simulink model "ElectricVehicleThermalManagementWithHeatPump_2026a_version"  (R2026a)
settings: Solver=VariableStepAuto  StopTime=3600  AbsTol=1e-3
PreLoadFcn:
  | init_nmpc
InitFcn:
  | init_nmpc
model workspace: external: MATLAB File ElectricVehicleThermalManagementWithHeatPumpParameters.m (data not in the file)
values from neighbouring files (symbols this model uses):
  battery_C1_LUT = [1913.6 12447 30609 ... (first row only)    [ElectricVehicleThermalManagementWithHeatPumpParameters.m]
  battery_capacity_LUT = [280.081 276.25 276.392]    [ElectricVehicleThermalManagementWithHeatPumpParameters.m]
  battery_cell_cp = 795    [ElectricVehicleThermalManagementWithHeatPumpParameters.m]
  battery_cell_mass = 2.5    [ElectricVehicleThermalManagementWithHeatPumpParameters.m]
  battery_Em_LUT = [3.4966 3.5057 3.5148 ... (first row only)    [ElectricVehicleThermalManagementWithHeatPumpParameters.m]
  battery_N_cells = 20    [ElectricVehicleThermalManagementWithHeatPumpParameters.m]
  battery_Qe_init = 0    [ElectricVehicleThermalManagementWithHeatPumpParameters.m]
  battery_R0_LUT = [0.0117 0.0085 0.009 ... (first row only)    [ElectricVehicleThermalManagementWithHeatPumpParameters.m]
  battery_R1_LUT = [0.0109 0.0029 0.0013 ... (first row only)    [ElectricVehicleThermalManagementWithHeatPumpParameters.m]
  battery_SOC_LUT = [0; 0.1; 0.25; 0.5; 0.75; 0.9; 1]    [ElectricVehicleThermalManagementWithHeatPumpParameters.m]
  battery_T_init = -5    [ElectricVehicleThermalManagementWithHeatPumpParameters.m]
  battery_temperature_LUT = [5 20 40]    [ElectricVehicleThermalManagementWithHeatPumpParameters.m]
  cabin_duct_area = 0.04    [ElectricVehicleThermalManagementWithHeatPumpParameters.m]
  cabin_T_init = -5    [ElectricVehicleThermalManagementWithHeatPumpParameters.m]
  chiller_area_primary = 0.43982297150257105    (= 0.439822971503)    [ElectricVehicleThermalManagementWithHeatPumpParameters.m]
  chiller_N_baffles = 3    [ElectricVehicleThermalManagementWithHeatPumpParameters.m]
  chiller_N_tubes = 100    [ElectricVehicleThermalManagementWithHeatPumpParameters.m]
  chiller_tube_D = 0.0035    [ElectricVehicleThermalManagementWithHeatPumpParameters.m]
  chiller_tube_L = 0.4    [ElectricVehicleThermalManagementWithHeatPumpParameters.m]
  chiller_wall_conductivity = 240    [ElectricVehicleThermalManagementWithHeatPumpParameters.m]
  chiller_wall_thickness = 0.0001    [ElectricVehicleThermalManagementWithHeatPumpParameters.m]
  cond_evap_air_area_flow = 0.3906    [ElectricVehicleThermalManagementWithHeatPumpParameters.m]
  cond_evap_air_area_primary = 1.4834999999999998    (= 1.4835)    [ElectricVehicleThermalManagementWithHeatPumpParameters.m]
  cond_evap_W = 0.015    [ElectricVehicleThermalManagementWithHeatPumpParameters.m]
  cond_evap_wall_conductivity = 240    [ElectricVehicleThermalManagementWithHeatPumpParameters.m]
  cond_evap_wall_thickness = 0.0001    [ElectricVehicleThermalManagementWithHeatPumpParameters.m]
  coolant_channel_D = 0.0092    [ElectricVehicleThermalManagementWithHeatPumpParameters.m]
  coolant_pipe_D = 0.019    [ElectricVehicleThermalManagementWithHeatPumpParameters.m]
  coolant_T_init = -5    [ElectricVehicleThermalManagementWithHeatPumpParameters.m]
  coolant_tank_area = 0.0121    [ElectricVehicleThermalManagementWithHeatPumpParameters.m]
  coolant_tank_volume = 1.25    [ElectricVehicleThermalManagementWithHeatPumpParameters.m]
  coolant_valve_D_ratio_max = 0.95    [ElectricVehicleThermalManagementWithHeatPumpParameters.m]
  coolant_valve_D_ratio_min = 0.001    [ElectricVehicleThermalManagementWithHeatPumpParameters.m]
  coolant_valve_displacement = 0.0063    [ElectricVehicleThermalManagementWithHeatPumpParameters.m]
  coolant_valve_S_max = 0.0053    [ElectricVehicleThermalManagementWithHeatPumpParameters.m]
  evaporator_air_area_flow = 0.12    [ElectricVehicleThermalManagementWithHeatPumpParameters.m]
  evaporator_air_area_primary = 0.4323    [ElectricVehicleThermalManagementWithHeatPumpParameters.m]
  evaporator_W = 0.015    [ElectricVehicleThermalManagementWithHeatPumpParameters.m]
  evaporator_wall_conductivity = 240    [ElectricVehicleThermalManagementWithHeatPumpParameters.m]
  evaporator_wall_thickness = 0.0001    [ElectricVehicleThermalManagementWithHeatPumpParameters.m]
  expansion_valve_D_ratio_max = 0.9    [ElectricVehicleThermalManagementWithHeatPumpParameters.m]
  hex_area_primary = 0.070371675440411369    (= 0.0703716754404)    [ElectricVehicleThermalManagementWithHeatPumpParameters.m]
  hex_N_tubes = 64    [ElectricVehicleThermalManagementWithHeatPumpParameters.m]
  hex_tube_D = 0.0035    [ElectricVehicleThermalManagementWithHeatPumpParameters.m]
  hex_wall_conductivity = 240    [ElectricVehicleThermalManagementWithHeatPumpParameters.m]
  hex_wall_thickness = 0.0001    [ElectricVehicleThermalManagementWithHeatPumpParameters.m]
  inner_cond_air_area_flow = 0.1953    [ElectricVehicleThermalManagementWithHeatPumpParameters.m]
  inner_cond_air_area_primary = 0.99520000000000008    (= 0.9952)    [ElectricVehicleThermalManagementWithHeatPumpParameters.m]
  inner_cond_W = 0.02    [ElectricVehicleThermalManagementWithHeatPumpParameters.m]
  inner_cond_wall_conductivity = 240    [ElectricVehicleThermalManagementWithHeatPumpParameters.m]
  inner_cond_wall_thickness = 0.0001    [ElectricVehicleThermalManagementWithHeatPumpParameters.m]
  pump_speed_max = 1000    [ElectricVehicleThermalManagementWithHeatPumpParameters.m]
  radiator_air_area_flow = 0.097499999999999989    (= 0.0975)    [ElectricVehicleThermalManagementWithHeatPumpParameters.m]
  radiator_air_area_primary = 0.43687499999999996    (= 0.436875)    [ElectricVehicleThermalManagementWithHeatPumpParameters.m]
  radiator_W = 0.015    [ElectricVehicleThermalManagementWithHeatPumpParameters.m]
  radiator_wall_conductivity = 240    [ElectricVehicleThermalManagementWithHeatPumpParameters.m]
  radiator_wall_thickness = 0.0001    [ElectricVehicleThermalManagementWithHeatPumpParameters.m]
  refrigerant_p_init = 0.25    [ElectricVehicleThermalManagementWithHeatPumpParameters.m]
  refrigerant_pipe_D = 0.01    [ElectricVehicleThermalManagementWithHeatPumpParameters.m]
  refrigerant_valve_D_ratio_max = 0.95    [ElectricVehicleThermalManagementWithHeatPumpParameters.m]
  refrigerant_valve_displacement = 0.005    [ElectricVehicleThermalManagementWithHeatPumpParameters.m]
libraries: fl_lib x227, nesl_utility x162, SimscapeFluids_lib x30, LiBatteryElements_lib x16, slpidlib x3, SignalEditorBlockLib x1
(part 5 of 13)

== system ElectricVehicleThermalManagementWithHeatPump_2026a_version/DCDC ==
  Controlled Heat Flow Rate Source : fl_lib/Thermal/Thermal Sources/Controlled Heat Flow Rate Source
  Coolant Jacket : SimscapeFluids_lib/Thermal Liquid/Pipes & Fittings/Pipe (TL)  dynamic_compressibility=simscape.enum.onoff.on  inertia=simscape.enum.onoff.off  num_segments=1  pipe_length=0.2 m  cross_section_geometry=fluids.thermal_liquid.pipes_fittings.enum.CrossSectionGeometry.Custom  pipe_diameter=0.1 m  pipe_inner_diameter=0.05 m  pipe_outer_diameter=0.1 m  pipe_width=0.1 m  pipe_height=0.1 m  pipe_major_axis=0.1 m  pipe_minor_axis=0.05 m  pipe_side=0.1 m  pipe_angle=30 deg  area=pi * coolant_channel_D^2 / 4 m^2  Dh=coolant_channel_D m  annular_heat_transfer_walls=fluids.thermal_liquid.pipes_fittings.enum.AnnularPipeWalls.AnnularInner  elevation_spec=foundation.enum.constant_variable.constant  elevation_gain=0 m  gravity_spec=foundation.enum.constant_variable.constant  g=9.81 m/s^2  pressure_loss_spec=fluids.thermal_liquid.pipes_fittings.enum.PressureLossSpec.Haaland  local_pressure_loss_spec=fluids.thermal_liquid.pipes_fittings.enum.LocalLossSpec.AggregateLength  length_add=0 m  loss_coefficient=0.1  roughness_spec=fluids.thermal_liquid.pipes_fittings.enum.RoughnessSpec.Custom  roughness=1.5e-5 m  Re_friction_TLU=[ 400 1000 1.5e+3 3e+3 4e+3 6e+3 1e+4 2e+4 4e+4 6e+4 1e+5 1e+8 ]  friction_factor_TLU=[ 0.264 0.112 0.07099999999999999 0.0417 0.0387 0.0268 0.025 0.0232 0.0226 0.022 0.0214 0.0214 ]  Re_lam=100  Re_tur=500  shape_factor=64  mdot_nominal=[ 0.1 1 ] kg/s  p_diff_nominal=[ 0.001 0.01 ] MPa  mdot_threshold=1e-6 kg/s  wall_spec=fluids.thermal_liquid.pipes_fittings.enum.wall_spec.rigid  vol_expansion_spec=fluids.thermal_liquid.pipes_fittings.enum.VolumeExpansionSpec.Diameter  area_pressure_gain=1e-6 m^2/MPa  static_pressure_TLU=[.1, 1] MPa  area_pressure_gain_TLU=[1e-05, 1.1e-05] m^2  material_behavior_spec=fluids.thermal_liquid.pipes_fittings.enum.PipeMaterialBehavior.Linear  diameter_pressure_gain=1.2e-6 m/MPa  wall_thickness=0.05 m  elastic_modulus=69 GPa  stress_TLU=[276, 310] MPa  strain_TLU=[.004, .02]  stress_assert_action=simscape.enum.assert.action.none  stress_max=400 MPa  poisson_ratio=0.33  wall_time_constant=0.01 s  environment_spec=foundation.enum.pressure_spec.atmospheric  environment_pressure=0.101325 MPa  thermal_expansion=false  alpha_L_wall=24 um/(deltaK*m)  thermal_expansion_Tref=293.15 K  heat_transfer_spec=fluids.thermal_liquid.pipes_fittings.enum.HeatTransferSpec.DittusBoelter  mdot_nominal_heat=[ 0.1 1 ] kg/s  T_in_nominal=[ 293.15 293.15 ] K  T_out_nominal=[ 300 300 ] K  p_in_nominal_heat=[ 0.101325 0.101325 ] MPa  T_wall_nominal=[ 303.15 303.15 ] K  T_wall_eff_nominal=[303.15, 303.15] K  a_coeff=0.3  b_Re_power=0.8  c_Pr_power=0.33  Nu_lam=3.66  Re_Colburn_TLU=[ 100 150 1000 ]  Colburn_factor_TLU=[ 0.019 0.013 0.002 ]  Re_Nu_TLU=[ 100 150 1000 ]  Pr_Nu_TLU=[ 1 10 ]  Nu_TLU=[ 3.72 4.21; 3.75 4.44; 4.21 7.15 ]  annular_correction=fluids.thermal_liquid.pipes_fittings.enum.AnnularPipeCorrectionFactor.Gnielinski  p0_vec=coolant_p_init MPa  T0_vec=coolant_T_init degC  mdot0=0.1 kg/s  p_nominal=0.101325 MPa  T_nominal=293.15 K
  DC-DC Converter : fl_lib/Thermal/Thermal Elements/Thermal Mass  mass_type=foundation.enum.constant_variable.constant  mass=1 kg  sp_heat=447 J/kg/K  mass_min=1e-6 kg  num_ports=foundation.enum.numPorts2.one  m_specify=off  m_priority=High  m=1 kg  m_nominal_specify=off  m_nominal_value=1  m_nominal_unit=kg  T_specify=on  T_priority=High  T=coolant_T_init degC  T_nominal_specify=off  T_nominal_value=1  T_nominal_unit=K  Q_specify=off  Q_priority=None  Q=0 W  Q_nominal_specify=off  Q_nominal_value=1  Q_nominal_unit=W
  Flow Rate Sensor (TL) : fl_lib/Thermal Liquid/Sensors/Flow Rate Sensor (TL)  mass_flow_measure=true  volumetric_flow_measure=false  energy_flow_measure=true
  Flow Resistance (TL) : fl_lib/Thermal Liquid/Elements/Flow Resistance (TL)  delta_p_nominal=2e-3 MPa  mdot_nominal=0.02 kg/s  area=pi * coolant_pipe_D^2 / 4 m^2  laminar_fraction=1e-3
  Flow Resistance (TL)1 : fl_lib/Thermal Liquid/Elements/Flow Resistance (TL)  delta_p_nominal=1e-5 MPa  mdot_nominal=0.02 kg/s  area=pi * coolant_pipe_D^2 / 4 m^2  laminar_fraction=1e-3
  PS-Simulink Converter : nesl_utility/PS-Simulink Converter  PhysicalDomain=network_engine_domain  SubClassName=ps_output  LeftPortType=input  RightPortType=output  PseudoPeriodic=off  Frequencies=[]  VectorFormat=inherit  Unit=degC  AffineConversion=on
  PS-Simulink Converter1 : nesl_utility/PS-Simulink Converter  PhysicalDomain=network_engine_domain  SubClassName=ps_output  LeftPortType=input  RightPortType=output  PseudoPeriodic=off  Frequencies=[]  VectorFormat=inherit  Unit=inherit  AffineConversion=off
  Scope : Scope
      settings: ActiveDisplayYMinimum=-0.0018  ActiveDisplayYMaximum=0.01621  DataLoggingVariableName=ScopeData8
  Simulink-PS Converter : nesl_utility/Simulink-PS Converter  PhysicalDomain=network_engine_domain  SubClassName=ps_input  LeftPortType=input  RightPortType=output  PseudoPeriodic=off  Frequencies=[]  NoiseDistribution=none  NoiseParameters=[]  Unit=W  AffineConversion=off  FilteringAndDerivatives=provide  SimscapeFilterOrder=1  InputFilterTimeConstant=0.001  UdotUserProvided=0
  Temperature Sensor : fl_lib/Thermal/Thermal Sensors/Temperature Sensor  temperature_measure=foundation.enum.MeasurementReference.absolute
  Thermal Reference : fl_lib/Thermal/Thermal Elements/Thermal Reference
  To Workspace : ToWorkspace  VariableName=mf_dcdc  SampleTime=-1
  To Workspace1 : ToWorkspace  VariableName=Q_dcdcMeasured  SampleTime=-1
  To Workspace2 : ToWorkspace  VariableName=T_dcdcMeas  SampleTime=-1
  B : PMIOPort  Side=Left
  A : PMIOPort  Port=2  Side=Right
  tag scope: T_dcdc=global
  wires:
  [Q_dcdc] -> To Workspace1/1, Simulink-PS Converter/1
  PS-Simulink Converter/1 -> To Workspace2/1, [T_dcdc]
  PS-Simulink Converter1/1 -> To Workspace/1, Scope/1
  connections:
  Coolant Jacket/LConn2 -- Controlled Heat Flow Rate Source/LConn1 -- Temperature Sensor/LConn1 -- DC-DC Converter/LConn1
  PS-Simulink Converter/LConn1 -- Temperature Sensor/RConn1
  Controlled Heat Flow Rate Source/RConn2 -- Thermal Reference/LConn1
  Simulink-PS Converter/RConn1 -- Controlled Heat Flow Rate Source/RConn1
  Coolant Jacket/LConn1 -- Flow Rate Sensor (TL)/RConn1
  PS-Simulink Converter1/LConn1 -- Flow Rate Sensor (TL)/RConn2
  Flow Resistance (TL)/LConn1 -- A/RConn1
  Flow Resistance (TL)/RConn1 -- Flow Rate Sensor (TL)/LConn1
  Flow Resistance (TL)1/LConn1 -- Coolant Jacket/RConn1
  Flow Resistance (TL)1/RConn1 -- B/RConn1

== system ElectricVehicleThermalManagementWithHeatPump_2026a_version/Evaporator ==
  Evaporator : SimscapeFluids_lib/Heat Exchangers/Two-Phase Fluid - Moist Air/Condenser Evaporator (2P-MA)  flow_arrangement=fluids.heat_exchangers.enum.FlowArrangement2PMA.Cross  cross_flow_arrangement=fluids.heat_exchangers.enum.CrossFlowArrangement2PMA.UnmixedUnmixed  R_wall=evaporator_wall_thickness / evaporator_air_area_primary / evaporator_wall_conductivity K/W  wall_thermal_mass=false  mass_wall=1 kg  cp_wall=490 J/(K*kg)  area_A1=pi * refrigerant_pipe_D^2 / 4 m^2  area_B1=pi * refrigerant_pipe_D^2 / 4 m^2  area_A2=cabin_duct_area m^2  area_B2=cabin_duct_area m^2  tube_num_2P=evaporator_N_tubes  tube_length_2P=evaporator_L m  tube_cross_section_2P=fluids.heat_exchangers.enum.TubeCrossSection.Rectangular  tube_diameter_2P=0.1 m  tube_width_2P=evaporator_W m  tube_height_2P=evaporator_tube_H m  tube_inner_diameter_2P=0.05 m  tube_outer_diameter_2P=0.1 m  tube_flow_area_2P=0.01 m^2  tube_wetted_perimeter_2P=0.4 m  tube_heat_perimeter_2P=0.4 m  tube_pressure_loss_spec_2P=fluids.heat_exchangers.enum.TubePressureLossSpec2P.Haaland  tube_loss_coeff_2P=10  tube_local_pressure_loss_spec_2P=fluids.heat_exchangers.enum.LocalLossSpec.AggregateLength  tube_length_add_2P=evaporator_tube_Leq m  tube_local_loss_coefficient_2P=0.1  tube_roughness_pressure_2P=15e-6 m  tube_Re_lam_pressure_2P=2000  tube_Re_tur_pressure_2P=4000  tube_shape_factor_generic_2P=64  tube_heat_coeff_spec_2P=fluids.heat_exchangers.enum.TubeHeatCoeffSpec2P.GneilinskiCavalliniZecchin  tube_colburn_coeff_liq_2P=[.023, .8, .33]  tube_colburn_coeff_mix_2P=[.05, .8, .33]  tube_colburn_coeff_vap_2P=[.023, .8, .33]  tube_roughness_heat_2P=15e-6 m  tube_Re_lam_heat_2P=2000  tube_Re_tur_heat_2P=4000  tube_Nu_lam_generic_2P=3.66  fouling_factor_2P=0.1 m^2*K/kW  fin_area_2P=evaporator_tube_area_webs m^2  fin_efficiency_2P=0.6  energy_spec_2P=foundation.enum.energy_spec.void_fraction  p_init_2P=refrigerant_p_init MPa  T_init_2P=293.15 K  x_init_2P=0.5  alpha_init_2P=refrigerant_alpha_init  h_init_2P=1500 kJ/kg  u_init_2P=1500 kJ/kg  flow_geometry_MA=fluids.heat_exchangers.enum.FlowGeometryMA.Generic  tube_num_MA=1  tube_length_MA=5 m  tube_cross_section_MA=fluids.heat_exchangers.enum.TubeCrossSection.Circular  tube_diameter_MA=0.1 m  tube_width_MA=0.1 m  tube_height_MA=0.1 m  tube_inner_diameter_MA=0.05 m  tube_outer_diameter_MA=0.1 m  tube_flow_area_MA=0.01 m^2  tube_wetted_perimeter_MA=0.4 m  tube_heat_perimeter_MA=0.4 m  tube_pressure_loss_spec_MA=fluids.heat_exchangers.enum.TubePressureLossSpec.Haaland  tube_loss_coeff_MA=10  tube_local_pressure_loss_spec_MA=fluids.heat_exchangers.enum.LocalLossSpec.AggregateLength  tube_length_add_MA=0.1 m  tube_local_loss_coefficient_MA=0.1  tube_roughness_pressure_MA=15e-6 m  tube_Re_lam_pressure_MA=2000  tube_Re_tur_pressure_MA=4000  tube_shape_factor_generic_MA=64  tube_heat_coeff_spec_MA=fluids.heat_exchangers.enum.TubeHeatCoeffSpec.Gneilinski  tube_colburn_coeff_MA=[.023, .8, .33]  tube_roughness_heat_MA=15e-6 m  tube_Re_lam_heat_MA=2000  tube_Re_tur_heat_MA=4000  tube_Nu_lam_generic_MA=3.66  bank_arrangement_MA=fluids.heat_exchangers.enum.BankArrangement.Inline  bank_num_rows_MA=5  bank_tubes_per_row_MA=5  bank_width_MA=1 m  bank_tube_diameter_MA=0.05 m  bank_longitudinal_pitch_MA=0.15 m  bank_transverse_pitch_MA=0.15 m  bank_pressure_loss_spec_MA=fluids.heat_exchangers.enum.BankPressureLossSpec.Martin  bank_euler_MA=10  bank_heat_coeff_spec_MA=fluids.heat_exchangers.enum.BankHeatCoeffSpec.Martin  bank_colburn_coeff_MA=[.27, .63, .36]  generic_flow_area_MA=evaporator_air_area_flow m^2  generic_heat_area_MA=evaporator_air_area_primary m^2  generic_volume_MA=evaporator_air_area_flow * evaporator_W m^3  generic_loss_coeff_MA=10  generic_colburn_coeff_MA=[0.27, 0.63, 0.36]  fouling_factor_MA=0.1 m^2*K/kW  fin_area_MA=evaporator_air_area_fins m^2  fin_efficiency_MA=0.7  p_init_MA=cabin_p_init MPa  T_init_MA=cabin_T_init degC  humidity_spec_MA=foundation.enum.HumiditySpec.RelativeHumidity  RH_init_MA=cabin_RH_init  x_w_init_MA=0.01  y_w_init_MA=0.01  HR_init_MA=0.01  Tw_init_MA=287 K  trace_gas_spec_MA=foundation.enum.trace_gas_spec.mole_fraction  x_g_init_MA=0.001  y_g_init_MA=cabin_CO2_init  r_d_init_MA=0  RH_ws_MA=1  time_constant_cond_MA=1e-3 s  time_constant_evap_MA=1e-3 s  fraction_entrained_MA=1
  Flow Resistance (2P) : fl_lib/Two-Phase Fluid/Elements/Flow Resistance (2P)  delta_p_nominal=1e-4 MPa  mdot_nominal=0.01 kg/s  v_nominal=0 m^3/kg  area=pi * refrigerant_pipe_D^2 / 4 m^2  laminar_fraction=1e-3
  PS-Simulink Converter{,1..3} (4 alike) : nesl_utility/PS-Simulink Converter  PhysicalDomain=network_engine_domain  SubClassName=ps_output  LeftPortType=input  RightPortType=output  PseudoPeriodic=off  Frequencies=[]  VectorFormat=inherit  Unit=inherit  AffineConversion=off
  Pressure & Temperature Sensor (MA) : fl_lib/Moist Air/Sensors/Pressure & Temperature Sensor (MA)  reference=foundation.enum.MeasurementReference.absolute  pressure=true  pressure_spec=foundation.enum.PressureMeasementSpec.Absolute  temperature=true
  Pressure & Temperature Sensor (MA)1 : fl_lib/Moist Air/Sensors/Pressure & Temperature Sensor (MA)  reference=foundation.enum.MeasurementReference.absolute  pressure=true  pressure_spec=foundation.enum.PressureMeasementSpec.Absolute  temperature=true
  SR7 : Subsystem
  SR8 : Subsystem
  Scope : Scope
      settings: ActiveDisplayYMinimum=254.07357  ActiveDisplayYMaximum=301.11104  DataLoggingVariableName=ScopeData3
  To Workspace : ToWorkspace  VariableName=airEvapPressure_out  SampleTime=-1
  To Workspace1 : ToWorkspace  VariableName=airEvapTemp_out  SampleTime=-1
  To Workspace2 : ToWorkspace  VariableName=airEvapPressure_in  SampleTime=-1
  To Workspace3 : ToWorkspace  VariableName=airEvapTemp_in  SampleTime=-1
  A : PMIOPort  Side=Left
  D : PMIOPort  Port=2  Side=Left
  B : PMIOPort  Port=3  Side=Right
  C : PMIOPort  Port=4  Side=Right
  wires:
  PS-Simulink Converter/1 -> To Workspace/1
  PS-Simulink Converter3/1 -> Scope/1, To Workspace1/1
  PS-Simulink Converter1/1 -> To Workspace2/1
  PS-Simulink Converter2/1 -> To Workspace3/1
  connections:
  SR8/LConn1 -- Evaporator/LConn3
  SR7/RConn1 -- Evaporator/LConn1
  SR8/RConn1 -- Flow Resistance (2P)/LConn1
  Evaporator/RConn3 -- Pressure & Temperature Sensor (MA)1/LConn1 -- C/RConn1
  Flow Resistance (2P)/RConn1 -- B/RConn1
  Evaporator/RConn1 -- D/RConn1 -- Pressure & Temperature Sensor (MA)/LConn1
  SR7/LConn1 -- A/RConn1
  PS-Simulink Converter/LConn1 -- Pressure & Temperature Sensor (MA)/RConn1
  PS-Simulink Converter1/LConn1 -- Pressure & Temperature Sensor (MA)1/RConn1
  PS-Simulink Converter2/LConn1 -- Pressure & Temperature Sensor (MA)1/RConn2
  PS-Simulink Converter3/LConn1 -- Pressure & Temperature Sensor (MA)/RConn2

== system ElectricVehicleThermalManagementWithHeatPump_2026a_version/Evaporator Expansion Valve ==
  Evaporator Expansion Valve : SimscapeFluids_lib/Two-Phase Fluid/Valves & Orifices/Orifice (2P)  orifice_type=foundation.enum.constant_variable.variable  constant_liquid_orifice_parameterization=fluids.two_phase_fluid.valves_orifices.enum.LiquidConstantOrificeParameterization.Area  variable_liquid_orifice_parameterization=fluids.two_phase_fluid.valves_orifices.enum.LiquidOrificeParameterization.LinearArea  mdot_nominal_constant=0.1 kg/s  delta_p_nominal_constant=0.001 MPa  orifice_area_constant=1e-4 m^2  S_min=0 m  del_S=refrigerant_valve_displacement m  open_orientation=fluids.two_phase_fluid.valves_orifices.enum.OrificeOrientation.Positive  mdot_nominal_max=0.1 kg/s  delta_p_nominal_max=0.001 MPa  orifice_area_max=pi * (expansion_valve_D_ratio_max*refrigerant_pipe_D)^2 / 4 m^2  S_TLU=[0, .002, .004, .007, .017] m  orifice_area_TLU=[1e-10, 2e-05, 4e-05, 6e-05, 8e-05, .0001] m^2  energy_spec=foundation.enum.energy_spec.temperature  p_inlet=0.101325 MPa  T_inlet=293.15 K  x_inlet=0  alpha_inlet=0  h_inlet=400 kJ/kg  u_inlet=400 kJ/kg  Cd=0.7  pressure_recovery=true  leakage_fraction=1e-6  smoothing_factor=0.01  B_lam=0.999  tau_x=0.1 s  area=pi * refrigerant_pipe_D^2 / 4 m^2  vapor_orifice_parameterization=fluids.two_phase_fluid.valves_orifices.enum.VaporOrificeParameterization.Cv  opening_characteristic=fluids.two_phase_fluid.valves_orifices.enum.OpeningCharacteristics.Linear  Cv_constant=4  Cv_max=4  S_Cv_TLU=[0, .003, .006, .009, .012, .015] m  Cv_TLU=[1e-06, .8, 1.6, 2.4, 3.2, 4]  xT_Cv=0.7  Kv_constant=3.6  Kv_max=3.6  S_Kv_TLU=[0, .003, .006, .009, .012, .015] m  Kv_TLU=[1e-06, .72, 1.44, 2.16, 2.88, 3.6]  xT_Kv=0.7  S_orifice_area_TLU=[0, .003, .006, .009, .012, .015] m
  Max Valve Displacement [m] : Gain  Gain=refrigerant_valve_displacement
  Simulink-PS Converter : nesl_utility/Simulink-PS Converter  PhysicalDomain=network_engine_domain  SubClassName=ps_input  LeftPortType=input  RightPortType=output  PseudoPeriodic=off  Frequencies=[]  NoiseDistribution=none  NoiseParameters=[]  Unit=m  AffineConversion=off  FilteringAndDerivatives=provide  SimscapeFilterOrder=1  InputFilterTimeConstant=0.001  UdotUserProvided=0
  Transfer Fcn : TransferFcn  Denominator=[1 1]
  A : PMIOPort  Side=Left
  B : PMIOPort  Port=2  Side=Right
  wires:
  Transfer Fcn/1 -> Max Valve Displacement [m]/1
  [cmd_exv_evap] -> Transfer Fcn/1
  Max Valve Displacement [m]/1 -> Simulink-PS Converter/1
  connections:
  Evaporator Expansion Valve/LConn2 -- Simulink-PS Converter/RConn1
  Evaporator Expansion Valve/LConn1 -- A/RConn1
  Evaporator Expansion Valve/RConn1 -- B/RConn1

== system ElectricVehicleThermalManagementWithHeatPump_2026a_version/Heat Exchanger ==
  Flow Rate Sensor (TL) : fl_lib/Thermal Liquid/Sensors/Flow Rate Sensor (TL)  mass_flow_measure=true  volumetric_flow_measure=false  energy_flow_measure=true
  Heat Exchanger : SimscapeFluids_lib/Heat Exchangers/Two-Phase Fluid - Thermal Liquid/Condenser Evaporator (TL-2P)  flow_arrangement=fluids.heat_exchangers.enum.FlowArrangementTL2P.Cross  cross_flow_arrangement=fluids.heat_exchangers.enum.CrossFlowArrangementTL2P.UnmixedMixed  R_wall=hex_wall_thickness / hex_area_primary / hex_wall_conductivity K/W  wall_thermal_mass=false  mass_wall=1 kg  cp_wall=490 J/(K*kg)  area_A1=pi * coolant_pipe_D^2 / 4 m^2  area_B1=pi * coolant_pipe_D^2 / 4 m^2  area_A2=pi * refrigerant_pipe_D^2 / 4 m^2  area_B2=pi * refrigerant_pipe_D^2 / 4 m^2  flow_geometry_TL=fluids.heat_exchangers.enum.FlowGeometryTL.AcrossTubeBank  tube_num_TL=1  tube_length_TL=5 m  tube_cross_section_TL=fluids.heat_exchangers.enum.TubeCrossSection.Circular  tube_diameter_TL=0.1 m  tube_width_TL=0.1 m  tube_height_TL=0.1 m  tube_inner_diameter_TL=0.05 m  tube_outer_diameter_TL=0.1 m  tube_flow_area_TL=0.01 m^2  tube_wetted_perimeter_TL=0.4 m  tube_heat_perimeter_TL=0.4 m  tube_pressure_loss_spec_TL=fluids.heat_exchangers.enum.TubePressureLossSpec.Haaland  tube_loss_coeff_TL=10  tube_local_pressure_loss_spec_TL=fluids.heat_exchangers.enum.LocalLossSpec.AggregateLength  tube_length_add_TL=0.1 m  tube_local_loss_coefficient_TL=0.1  tube_roughness_pressure_TL=15e-6 m  tube_Re_lam_pressure_TL=2000  tube_Re_tur_pressure_TL=4000  tube_shape_factor_generic_TL=64  tube_heat_coeff_spec_TL=fluids.heat_exchangers.enum.TubeHeatCoeffSpec.Gneilinski  tube_colburn_coeff_TL=[.023, .8, .33]  tube_roughness_heat_TL=15e-6 m  tube_Re_lam_heat_TL=2000  tube_Re_tur_heat_TL=4000  tube_Nu_lam_generic_TL=3.66  bank_arrangement_TL=fluids.heat_exchangers.enum.BankArrangement.Staggered  bank_num_rows_TL=sqrt(hex_N_tubes)  bank_tubes_per_row_TL=sqrt(hex_N_tubes)  bank_width_TL=hex_tube_L m  bank_tube_diameter_TL=hex_tube_D m  bank_longitudinal_pitch_TL=2 * hex_tube_D m  bank_transverse_pitch_TL=2 * hex_tube_D m  bank_pressure_loss_spec_TL=fluids.heat_exchangers.enum.BankPressureLossSpec.Martin  bank_euler_TL=10  bank_heat_coeff_spec_TL=fluids.heat_exchangers.enum.BankHeatCoeffSpec.Martin  bank_colburn_coeff_TL=[.27, .63, .36]  generic_flow_area_TL=0.01 m^2  generic_heat_area_TL=2 m^2  generic_volume_TL=0.05 m^3  generic_loss_coeff_TL=10  generic_colburn_coeff_TL=[.023, .8, .33]  fouling_factor_TL=0.1 m^2*K/kW  fin_area_TL=0 m^2  fin_efficiency_TL=0  p_init_TL=coolant_p_init MPa  T_init_TL=coolant_T_init degC  tube_num_2P=hex_N_tubes  tube_length_2P=hex_tube_L m  tube_cross_section_2P=fluids.heat_exchangers.enum.TubeCrossSection.Circular  tube_diameter_2P=hex_tube_D m  tube_width_2P=0.1 m  tube_height_2P=0.1 m  tube_inner_diameter_2P=0.05 m  tube_outer_diameter_2P=0.1 m  tube_flow_area_2P=0.01 m^2  tube_wetted_perimeter_2P=0.4 m  tube_heat_perimeter_2P=0.4 m  tube_pressure_loss_spec_2P=fluids.heat_exchangers.enum.TubePressureLossSpec2P.Haaland  tube_loss_coeff_2P=10  tube_local_pressure_loss_spec_2P=fluids.heat_exchangers.enum.LocalLossSpec.AggregateLength  tube_length_add_2P=hex_tube_Leq m  tube_local_loss_coefficient_2P=0.1  tube_roughness_pressure_2P=15e-6 m  tube_Re_lam_pressure_2P=2000  tube_Re_tur_pressure_2P=4000  tube_shape_factor_generic_2P=64  tube_heat_coeff_spec_2P=fluids.heat_exchangers.enum.TubeHeatCoeffSpec2P.GneilinskiCavalliniZecchin  tube_colburn_coeff_liq_2P=[.023, .8, .33]  tube_colburn_coeff_mix_2P=[.05, .8, .33]  tube_colburn_coeff_vap_2P=[.023, .8, .33]  tube_roughness_heat_2P=15e-6 m  tube_Re_lam_heat_2P=2000  tube_Re_tur_heat_2P=4000  tube_Nu_lam_generic_2P=3.66  fouling_factor_2P=0.1 m^2*K/kW  fin_area_2P=0 m^2  fin_efficiency_2P=0  energy_spec_2P=foundation.enum.energy_spec.void_fraction  p_init_2P=refrigerant_p_init MPa  T_init_2P=293.15 K  x_init_2P=0.5  alpha_init_2P=refrigerant_alpha_init  h_init_2P=1500 kJ/kg  u_init_2P=1500 kJ/kg
  PS-Simulink Converter : nesl_utility/PS-Simulink Converter  PhysicalDomain=network_engine_domain  SubClassName=ps_output  LeftPortType=input  RightPortType=output  PseudoPeriodic=off  Frequencies=[]  VectorFormat=inherit  Unit=inherit  AffineConversion=off
  PS-Simulink Converter1 : nesl_utility/PS-Simulink Converter  PhysicalDomain=network_engine_domain  SubClassName=ps_output  LeftPortType=input  RightPortType=output  PseudoPeriodic=off  Frequencies=[]  VectorFormat=inherit  Unit=inherit  AffineConversion=off
  PS-Simulink Converter2 : nesl_utility/PS-Simulink Converter  PhysicalDomain=network_engine_domain  SubClassName=ps_output  LeftPortType=input  RightPortType=output  PseudoPeriodic=off  Frequencies=[]  VectorFormat=inherit  Unit=inherit  AffineConversion=off
  Pressure & Temperature Sensor (TL) : fl_lib/Thermal Liquid/Sensors/Pressure & Temperature Sensor (TL)  reference=foundation.enum.MeasurementReference.absolute  pressure=false  pressure_spec=foundation.enum.PressureMeasementSpec.Absolute  temperature=true
  Pressure & Temperature Sensor (TL)1 : fl_lib/Thermal Liquid/Sensors/Pressure & Temperature Sensor (TL)  reference=foundation.enum.MeasurementReference.absolute  pressure=false  pressure_spec=foundation.enum.PressureMeasementSpec.Absolute  temperature=true
  SR5 : Subsystem
  SR6 : Subsystem
  Scope : Scope
      settings: ActiveDisplayYMinimum=256.69677  ActiveDisplayYMaximum=319.19994  DataLoggingVariableName=ScopeData2
  Scope1 : Scope
      settings: ActiveDisplayYMinimum=252.53888  ActiveDisplayYMaximum=358.65007  DataLoggingVariableName=ScopeData3
  Scope2 : Scope
      settings: ActiveDisplayYMinimum=-0.04462  ActiveDisplayYMaximum=0.40154
  To Workspace : ToWorkspace  VariableName=heatExchangerCoolantT_outK  SampleTime=-1
  To Workspace1 : ToWorkspace  VariableName=heatExchangerCoolantT_inK  SampleTime=-1
  To Workspace2 : ToWorkspace  VariableName=mf_htxClnt  SampleTime=-1
  D : PMIOPort  Side=Left
  A : PMIOPort  Port=2  Side=Left
  C : PMIOPort  Port=3  Side=Right
  B : PMIOPort  Port=4  Side=Right
  wires:
  PS-Simulink Converter/1 -> To Workspace/1, Scope/1
  PS-Simulink Converter1/1 -> Scope1/1, To Workspace1/1
  PS-Simulink Converter2/1 -> To Workspace2/1, Scope2/1
  connections:
  Heat Exchanger/RConn2 -- SR6/LConn1
  SR6/RConn1 -- B/RConn1
  Heat Exchanger/RConn1 -- SR5/RConn1
  SR5/LConn1 -- A/RConn1
  C/RConn1 -- Pressure & Temperature Sensor (TL)1/LConn1 -- Heat Exchanger/LConn2
  Pressure & Temperature Sensor (TL)/LConn1 -- D/RConn1 -- Flow Rate Sensor (TL)/RConn1
  PS-Simulink Converter/LConn1 -- Pressure & Temperature Sensor (TL)/RConn1
  PS-Simulink Converter1/LConn1 -- Pressure & Temperature Sensor (TL)1/RConn1
  PS-Simulink Converter2/LConn1 -- Flow Rate Sensor (TL)/RConn2
  Flow Rate Sensor (TL)/LConn1 -- Heat Exchanger/LConn1

== system ElectricVehicleThermalManagementWithHeatPump_2026a_version/Heat Pump Expansion Valve ==
  Heat Pump Expansion Valve : SimscapeFluids_lib/Two-Phase Fluid/Valves & Orifices/Orifice (2P)  orifice_type=foundation.enum.constant_variable.variable  constant_liquid_orifice_parameterization=fluids.two_phase_fluid.valves_orifices.enum.LiquidConstantOrificeParameterization.Area  variable_liquid_orifice_parameterization=fluids.two_phase_fluid.valves_orifices.enum.LiquidOrificeParameterization.LinearArea  mdot_nominal_constant=0.1 kg/s  delta_p_nominal_constant=0.001 MPa  orifice_area_constant=1e-4 m^2  S_min=0 m  del_S=refrigerant_valve_displacement m  open_orientation=fluids.two_phase_fluid.valves_orifices.enum.OrificeOrientation.Positive  mdot_nominal_max=0.1 kg/s  delta_p_nominal_max=0.001 MPa  orifice_area_max=pi * (expansion_valve_D_ratio_max*refrigerant_pipe_D)^2 / 4 m^2  S_TLU=[0, .002, .004, .007, .017] m  orifice_area_TLU=[1e-10, 2e-05, 4e-05, 6e-05, 8e-05, .0001] m^2  energy_spec=foundation.enum.energy_spec.temperature  p_inlet=0.101325 MPa  T_inlet=293.15 K  x_inlet=0  alpha_inlet=0  h_inlet=400 kJ/kg  u_inlet=400 kJ/kg  Cd=0.7  pressure_recovery=true  leakage_fraction=1e-6  smoothing_factor=0.01  B_lam=0.999  tau_x=0.1 s  area=pi * refrigerant_pipe_D^2 / 4 m^2  vapor_orifice_parameterization=fluids.two_phase_fluid.valves_orifices.enum.VaporOrificeParameterization.Cv  opening_characteristic=fluids.two_phase_fluid.valves_orifices.enum.OpeningCharacteristics.Linear  Cv_constant=4  Cv_max=4  S_Cv_TLU=[0, .003, .006, .009, .012, .015] m  Cv_TLU=[1e-06, .8, 1.6, 2.4, 3.2, 4]  xT_Cv=0.7  Kv_constant=3.6  Kv_max=3.6  S_Kv_TLU=[0, .003, .006, .009, .012, .015] m  Kv_TLU=[1e-06, .72, 1.44, 2.16, 2.88, 3.6]  xT_Kv=0.7  S_orifice_area_TLU=[0, .003, .006, .009, .012, .015] m
  Max Valve Displacement [m] : Gain  Gain=refrigerant_valve_displacement
  PS-Simulink Converter : nesl_utility/PS-Simulink Converter  PhysicalDomain=network_engine_domain  SubClassName=ps_output  LeftPortType=input  RightPortType=output  PseudoPeriodic=off  Frequencies=[]  VectorFormat=inherit  Unit=inherit  AffineConversion=off
  PS-Simulink Converter1 : nesl_utility/PS-Simulink Converter  PhysicalDomain=network_engine_domain  SubClassName=ps_output  LeftPortType=input  RightPortType=output  PseudoPeriodic=off  Frequencies=[]  VectorFormat=inherit  Unit=inherit  AffineConversion=off
  "Pressure, Temperature & Internal Energy Sensor (2P)" : fl_lib/Two-Phase Fluid/Sensors/Pressure, Temperature & Internal Energy Sensor (2P)  reference=foundation.enum.MeasurementReference.absolute  pressure=true  pressure_spec=foundation.enum.PressureMeasementSpec.Absolute  temperature=false  internal_energy=false
  "Pressure, Temperature & Internal Energy Sensor (2P)1" : fl_lib/Two-Phase Fluid/Sensors/Pressure, Temperature & Internal Energy Sensor (2P)  reference=foundation.enum.MeasurementReference.absolute  pressure=true  pressure_spec=foundation.enum.PressureMeasementSpec.Absolute  temperature=false  internal_energy=false
  Scope : Scope
      settings: ActiveDisplayYMinimum=-4E-6  ActiveDisplayYMaximum=3.9E-5
  Simulink-PS Converter : nesl_utility/Simulink-PS Converter  PhysicalDomain=network_engine_domain  SubClassName=ps_input  LeftPortType=input  RightPortType=output  PseudoPeriodic=off  Frequencies=[]  NoiseDistribution=none  NoiseParameters=[]  Unit=m  AffineConversion=off  FilteringAndDerivatives=provide  SimscapeFilterOrder=1  InputFilterTimeConstant=0.001  UdotUserProvided=0
  To Workspace : ToWorkspace  VariableName=EXVRefPress_inMpa  SampleTime=-1
  To Workspace1 : ToWorkspace  VariableName=EXVRefPress_outMpa  SampleTime=-1
  Transfer Fcn : TransferFcn  Denominator=[1 1]
  B : PMIOPort  Side=Left
  A : PMIOPort  Port=2  Side=Right
  wires:
  Max Valve Displacement [m]/1 -> Scope/1, Simulink-PS Converter/1
  [cmd_exv_heatpump] -> Transfer Fcn/1
  Transfer Fcn/1 -> Max Valve Displacement [m]/1
  PS-Simulink Converter/1 -> To Workspace/1
  PS-Simulink Converter1/1 -> To Workspace1/1
  connections:
  Heat Pump Expansion Valve/RConn1 -- "Pressure, Temperature & Internal Energy Sensor (2P)1"/LConn1 -- B/RConn1
  Heat Pump Expansion Valve/LConn1 -- "Pressure, Temperature & Internal Energy Sensor (2P)"/LConn1 -- A/RConn1
  Heat Pump Expansion Valve/LConn2 -- Simulink-PS Converter/RConn1
  PS-Simulink Converter/LConn1 -- "Pressure, Temperature & Internal Energy Sensor (2P)"/RConn1
  PS-Simulink Converter1/LConn1 -- "Pressure, Temperature & Internal Energy Sensor (2P)1"/RConn1

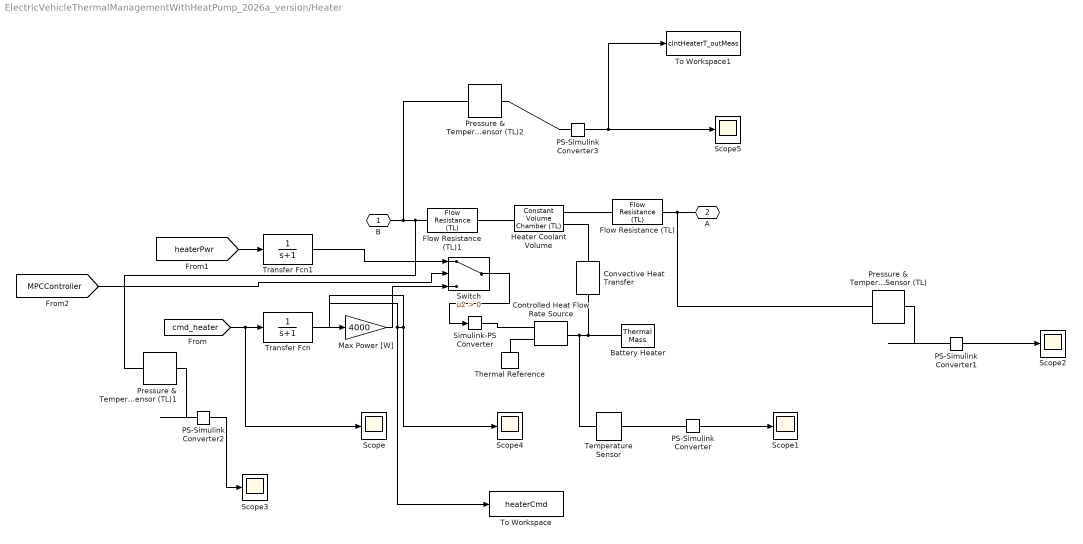
== system ElectricVehicleThermalManagementWithHeatPump_2026a_version/Heater ==
  Battery Heater : fl_lib/Thermal/Thermal Elements/Thermal Mass  mass_type=foundation.enum.constant_variable.constant  mass=2 kg  sp_heat=447 J/kg/K  mass_min=1e-6 kg  num_ports=foundation.enum.numPorts2.one  m_specify=off  m_priority=High  m=1 kg  m_nominal_specify=off  m_nominal_value=1  m_nominal_unit=kg  T_specify=on  T_priority=High  T=coolant_T_init degC  T_nominal_specify=off  T_nominal_value=1  T_nominal_unit=K  Q_specify=off  Q_priority=None  Q=0 W  Q_nominal_specify=off  Q_nominal_value=1  Q_nominal_unit=W
  Controlled Heat Flow Rate Source : fl_lib/Thermal/Thermal Sources/Controlled Heat Flow Rate Source
  Convective Heat Transfer : fl_lib/Thermal/Thermal Elements/Convective Heat Transfer  thermal_type=foundation.enum.constant_variable.constant  area=1 m^2  heat_tr_coeff=200 W/(m^2 * K)  min_heat_tr_coeff=1e-3 W/(K*m^2)  T_specify=off  T_priority=None  T=0 K  T_nominal_specify=off  T_nominal_value=1  T_nominal_unit=K  Q_specify=off  Q_priority=None  Q=0 W  Q_nominal_specify=off  Q_nominal_value=1  Q_nominal_unit=W
  Flow Resistance (TL) : fl_lib/Thermal Liquid/Elements/Flow Resistance (TL)  delta_p_nominal=2e-4 MPa  mdot_nominal=0.15 kg/s  area=pi * coolant_pipe_D^2 / 4 m^2  laminar_fraction=1e-3
  Flow Resistance (TL)1 : fl_lib/Thermal Liquid/Elements/Flow Resistance (TL)  delta_p_nominal=2e-4 MPa  mdot_nominal=0.15 kg/s  area=pi * coolant_pipe_D^2 / 4 m^2  laminar_fraction=1e-3
  Heater Coolant Volume : fl_lib/Thermal Liquid/Elements/Constant Volume Chamber (TL)  volume=0.001 m^3  num_ports=foundation.enum.num_ports.two  area_A=pi * coolant_pipe_D^2 / 4 m^2  area_B=pi * coolant_pipe_D^2 / 4 m^2  area_C=0.01 m^2  area_D=0.01 m^2  p_I_specify=on  p_I_priority=High  p_I=coolant_p_init MPa  p_I_nominal_specify=off  p_I_nominal_value=1  p_I_nominal_unit=MPa  T_I_specify=on  T_I_priority=High  T_I=coolant_T_init degC  T_I_nominal_specify=off  T_I_nominal_value=1  T_I_nominal_unit=K  u_I_specify=off  u_I_priority=None  u_I=83.90600000000001 kJ/kg  u_I_nominal_specify=off  u_I_nominal_value=1  u_I_nominal_unit=kJ/kg  rho_I_specify=off  rho_I_priority=None  rho_I=998.21 kg/m^3  rho_I_nominal_specify=off  rho_I_nominal_value=1  rho_I_nominal_unit=kg/m^3
  Max Power [W] : Gain  Gain=4000
  PS-Simulink Converter{,1..3} (4 alike) : nesl_utility/PS-Simulink Converter  PhysicalDomain=network_engine_domain  SubClassName=ps_output  LeftPortType=input  RightPortType=output  PseudoPeriodic=off  Frequencies=[]  VectorFormat=inherit  Unit=inherit  AffineConversion=off
  Pressure & Temperature Sensor (TL) : fl_lib/Thermal Liquid/Sensors/Pressure & Temperature Sensor (TL)  reference=foundation.enum.MeasurementReference.absolute  pressure=false  pressure_spec=foundation.enum.PressureMeasementSpec.Absolute  temperature=true
  Pressure & Temperature Sensor (TL)1 : fl_lib/Thermal Liquid/Sensors/Pressure & Temperature Sensor (TL)  reference=foundation.enum.MeasurementReference.absolute  pressure=false  pressure_spec=foundation.enum.PressureMeasementSpec.Absolute  temperature=true
  Pressure & Temperature Sensor (TL)2 : fl_lib/Thermal Liquid/Sensors/Pressure & Temperature Sensor (TL)  reference=foundation.enum.MeasurementReference.absolute  pressure=false  pressure_spec=foundation.enum.PressureMeasementSpec.Absolute  temperature=true
  Scope{,1..5} (6 alike) : Scope
      Scope settings: ActiveDisplayYMinimum=-0.125  ActiveDisplayYMaximum=1.125  DataLoggingVariableName=ScopeData3
      Scope1 settings: ActiveDisplayYMinimum=257.54019  ActiveDisplayYMaximum=313.63829
      Scope2 settings: ActiveDisplayYMinimum=266.52382  ActiveDisplayYMaximum=286.17075  DataLoggingVariableName=ScopeData2
      Scope3 settings: ActiveDisplayYMinimum=277.38138  ActiveDisplayYMaximum=289.06324  DataLoggingVariableName=ScopeData3
      Scope4 settings: ActiveDisplayYMinimum=-0.125  ActiveDisplayYMaximum=1.125  DataLoggingVariableName=ScopeData4
      Scope5 settings: ActiveDisplayYMinimum=277.38138  ActiveDisplayYMaximum=289.06324  DataLoggingVariableName=ScopeData5
  Simulink-PS Converter : nesl_utility/Simulink-PS Converter  PhysicalDomain=network_engine_domain  SubClassName=ps_input  LeftPortType=input  RightPortType=output  PseudoPeriodic=off  Frequencies=[]  NoiseDistribution=none  NoiseParameters=[]  Unit=1  AffineConversion=off  FilteringAndDerivatives=provide  SimscapeFilterOrder=1  InputFilterTimeConstant=0.001  UdotUserProvided=0
  Switch : Switch  Criteria=u2 > Threshold  SaturateOnIntegerOverflow=off  InputSameDT=off
  Temperature Sensor : fl_lib/Thermal/Thermal Sensors/Temperature Sensor  temperature_measure=foundation.enum.MeasurementReference.absolute
  Thermal Reference : fl_lib/Thermal/Thermal Elements/Thermal Reference
  To Workspace : ToWorkspace  VariableName=heaterCmd  SampleTime=-1
  To Workspace1 : ToWorkspace  VariableName=clntHeaterT_outMeas  SampleTime=-1
  Transfer Fcn : TransferFcn  Denominator=[1 1]
  Transfer Fcn1 : TransferFcn  Denominator=[1 1]
  B : PMIOPort  Side=Left
  A : PMIOPort  Port=2  Side=Right
  wires:
  [cmd_heater] -> Scope/1, Transfer Fcn/1
  Transfer Fcn/1 -> To Workspace/1, Scope4/1, Max Power [W]/1
  PS-Simulink Converter/1 -> Scope1/1
  PS-Simulink Converter1/1 -> Scope2/1
  PS-Simulink Converter2/1 -> Scope3/1
  PS-Simulink Converter3/1 -> To Workspace1/1, Scope5/1
  [heaterPwr] -> Transfer Fcn1/1
  Max Power [W]/1 -> Switch/3
  Transfer Fcn1/1 -> Switch/1
  [MPCController] -> Switch/2
  Switch/1 -> Simulink-PS Converter/1
  connections:
  Battery Heater/LConn1 -- Temperature Sensor/LConn1 -- Controlled Heat Flow Rate Source/LConn1 -- Convective Heat Transfer/LConn1
  Convective Heat Transfer/RConn1 -- Heater Coolant Volume/LConn2
  Flow Resistance (TL)/LConn1 -- Pressure & Temperature Sensor (TL)/LConn1 -- A/RConn1
  Flow Resistance (TL)1/RConn1 -- Pressure & Temperature Sensor (TL)1/LConn1 -- Pressure & Temperature Sensor (TL)2/LConn1 -- B/RConn1
  Flow Resistance (TL)1/LConn1 -- Heater Coolant Volume/RConn1
  Flow Resistance (TL)/RConn1 -- Heater Coolant Volume/LConn1
  Thermal Reference/LConn1 -- Controlled Heat Flow Rate Source/RConn2
  Temperature Sensor/RConn1 -- PS-Simulink Converter/LConn1
  PS-Simulink Converter1/LConn1 -- Pressure & Temperature Sensor (TL)/RConn1
  PS-Simulink Converter2/LConn1 -- Pressure & Temperature Sensor (TL)1/RConn1
  PS-Simulink Converter3/LConn1 -- Pressure & Temperature Sensor (TL)2/RConn1
  Simulink-PS Converter/RConn1 -- Controlled Heat Flow Rate Source/RConn1

== system ElectricVehicleThermalManagementWithHeatPump_2026a_version/Inner Condenser ==
  Flow Rate Sensor (MA) : fl_lib/Moist Air/Sensors/Flow Rate Sensor (MA)  mass_flow_measure=true  volumetric_flow_measure=false  volumetric_flow_conditions=foundation.enum.volumetric_flow_conditions.actual  p_std=0.101325 MPa  T_std=20 degC  humidity_spec=foundation.enum.HumiditySpec.RelativeHumidity  RH_std=0.65  x_w_std=0.01  y_w_std=0.01  HR_std=0.01  Tw_std=287 K  trace_gas_spec=foundation.enum.trace_gas_spec.mass_fraction  x_g_std=0  y_g_std=0  RH_ws=1  energy_flow_measure=true  vapor_flow_measure=false  gas_flow_measure=false  droplets_flow_measure=false
  Inner Condenser : SimscapeFluids_lib/Heat Exchangers/Two-Phase Fluid - Moist Air/Condenser Evaporator (2P-MA)  flow_arrangement=fluids.heat_exchangers.enum.FlowArrangement2PMA.Cross  cross_flow_arrangement=fluids.heat_exchangers.enum.CrossFlowArrangement2PMA.UnmixedUnmixed  R_wall=inner_cond_wall_thickness / inner_cond_air_area_primary / inner_cond_wall_conductivity K/kW  wall_thermal_mass=false  mass_wall=1 kg  cp_wall=490 J/(K*kg)  area_A1=pi * refrigerant_pipe_D^2 / 4 m^2  area_B1=pi * refrigerant_pipe_D^2 / 4 m^2  area_A2=cabin_duct_area m^2  area_B2=cabin_duct_area m^2  tube_num_2P=inner_cond_N_tubes  tube_length_2P=inner_cond_L m  tube_cross_section_2P=fluids.heat_exchangers.enum.TubeCrossSection.Rectangular  tube_diameter_2P=0.05 m  tube_width_2P=inner_cond_W m  tube_height_2P=inner_cond_tube_H m  tube_inner_diameter_2P=0.05 m  tube_outer_diameter_2P=0.1 m  tube_flow_area_2P=0.002 m^2  tube_wetted_perimeter_2P=0.15 m  tube_heat_perimeter_2P=0.15 m  tube_pressure_loss_spec_2P=fluids.heat_exchangers.enum.TubePressureLossSpec2P.Haaland  tube_loss_coeff_2P=10  tube_local_pressure_loss_spec_2P=fluids.heat_exchangers.enum.LocalLossSpec.AggregateLength  tube_length_add_2P=inner_cond_tube_Leq m  tube_local_loss_coefficient_2P=0.1  tube_roughness_pressure_2P=15e-6 m  tube_Re_lam_pressure_2P=2000  tube_Re_tur_pressure_2P=4000  tube_shape_factor_generic_2P=64  tube_heat_coeff_spec_2P=fluids.heat_exchangers.enum.TubeHeatCoeffSpec2P.GneilinskiCavalliniZecchin  tube_colburn_coeff_liq_2P=[.023, .8, .33]  tube_colburn_coeff_mix_2P=[.05, .8, .33]  tube_colburn_coeff_vap_2P=[.023, .8, .33]  tube_roughness_heat_2P=15e-6 m  tube_Re_lam_heat_2P=2000  tube_Re_tur_heat_2P=4000  tube_Nu_lam_generic_2P=3.66  fouling_factor_2P=0.1 K*m^2/kW  fin_area_2P=inner_cond_tube_area_webs m^2  fin_efficiency_2P=0.6  energy_spec_2P=foundation.enum.energy_spec.void_fraction  p_init_2P=refrigerant_p_init MPa  T_init_2P=293.15 K  x_init_2P=0.5  alpha_init_2P=refrigerant_alpha_init  h_init_2P=1500 kJ/kg  u_init_2P=1500 kJ/kg  flow_geometry_MA=fluids.heat_exchangers.enum.FlowGeometryMA.Generic  tube_num_MA=25  tube_length_MA=1 m  tube_cross_section_MA=fluids.heat_exchangers.enum.TubeCrossSection.Circular  tube_diameter_MA=0.05 m  tube_width_MA=0.05 m  tube_height_MA=0.05 m  tube_inner_diameter_MA=0.05 m  tube_outer_diameter_MA=0.1 m  tube_flow_area_MA=0.002 m^2  tube_wetted_perimeter_MA=0.15 m  tube_heat_perimeter_MA=0.15 m  tube_pressure_loss_spec_MA=fluids.heat_exchangers.enum.TubePressureLossSpec.Haaland  tube_loss_coeff_MA=10  tube_local_pressure_loss_spec_MA=fluids.heat_exchangers.enum.LocalLossSpec.AggregateLength  tube_length_add_MA=0.1 m  tube_local_loss_coefficient_MA=0.1  tube_roughness_pressure_MA=15e-6 m  tube_Re_lam_pressure_MA=2000  tube_Re_tur_pressure_MA=4000  tube_shape_factor_generic_MA=64  tube_heat_coeff_spec_MA=fluids.heat_exchangers.enum.TubeHeatCoeffSpec.Gneilinski  tube_colburn_coeff_MA=[.023, .8, .33]  tube_roughness_heat_MA=15e-6 m  tube_Re_lam_heat_MA=2000  tube_Re_tur_heat_MA=4000  tube_Nu_lam_generic_MA=3.66  bank_arrangement_MA=fluids.heat_exchangers.enum.BankArrangement.Inline  bank_num_rows_MA=5  bank_tubes_per_row_MA=5  bank_width_MA=1 m  bank_tube_diameter_MA=0.05 m  bank_longitudinal_pitch_MA=0.15 m  bank_transverse_pitch_MA=0.15 m  bank_pressure_loss_spec_MA=fluids.heat_exchangers.enum.BankPressureLossSpec.Martin  bank_euler_MA=10  bank_heat_coeff_spec_MA=fluids.heat_exchangers.enum.BankHeatCoeffSpec.Martin  bank_colburn_coeff_MA=[.27, .63, .36]  generic_flow_area_MA=inner_cond_air_area_flow m^2  generic_heat_area_MA=inner_cond_air_area_primary m^2  generic_volume_MA=inner_cond_air_area_flow * inner_cond_W m^3  generic_loss_coeff_MA=10  generic_colburn_coeff_MA=[.023, .8, .33]  fouling_factor_MA=0.1 K*m^2/kW  fin_area_MA=inner_cond_air_area_fins m^2  fin_efficiency_MA=0.7  p_init_MA=cabin_p_init MPa  T_init_MA=cabin_T_init degC  humidity_spec_MA=foundation.enum.HumiditySpec.RelativeHumidity  RH_init_MA=cabin_RH_init  x_w_init_MA=0.01  y_w_init_MA=0.01  HR_init_MA=0.01  Tw_init_MA=287 K  trace_gas_spec_MA=foundation.enum.trace_gas_spec.mole_fraction  x_g_init_MA=0.001  y_g_init_MA=cabin_CO2_init  r_d_init_MA=0  RH_ws_MA=1  time_constant_cond_MA=1e-3 s  time_constant_evap_MA=1e-3 s  fraction_entrained_MA=1
  PS-Simulink Converter : nesl_utility/PS-Simulink Converter  PhysicalDomain=network_engine_domain  SubClassName=ps_output  LeftPortType=input  RightPortType=output  PseudoPeriodic=off  Frequencies=[]  VectorFormat=inherit  Unit=inherit  AffineConversion=off
  PS-Simulink Converter1 : nesl_utility/PS-Simulink Converter  PhysicalDomain=network_engine_domain  SubClassName=ps_output  LeftPortType=input  RightPortType=output  PseudoPeriodic=off  Frequencies=[]  VectorFormat=inherit  Unit=inherit  AffineConversion=off
  PS-Simulink Converter2 : nesl_utility/PS-Simulink Converter  PhysicalDomain=network_engine_domain  SubClassName=ps_output  LeftPortType=input  RightPortType=output  PseudoPeriodic=off  Frequencies=[]  VectorFormat=inherit  Unit=inherit  AffineConversion=off
  Pressure & Temperature Sensor (MA) : fl_lib/Moist Air/Sensors/Pressure & Temperature Sensor (MA)  reference=foundation.enum.MeasurementReference.absolute  pressure=false  pressure_spec=foundation.enum.PressureMeasementSpec.Absolute  temperature=true
  Pressure & Temperature Sensor (MA)1 : fl_lib/Moist Air/Sensors/Pressure & Temperature Sensor (MA)  reference=foundation.enum.MeasurementReference.absolute  pressure=false  pressure_spec=foundation.enum.PressureMeasementSpec.Absolute  temperature=true
  SR1 : Subsystem
  SR2 : Subsystem
  Scope : Scope
      settings: ActiveDisplayYMinimum=-0.02165  ActiveDisplayYMaximum=0.19488  DataLoggingVariableName=ScopeData4
  Scope1 : Scope
      settings: ActiveDisplayYMinimum=262.40036  ActiveDisplayYMaximum=269.34475  DataLoggingVariableName=ScopeData17
  Scope2 : Scope
      settings: ActiveDisplayYMinimum=262.40542  ActiveDisplayYMaximum=263.23273  DataLoggingVariableName=ScopeData18
  To Workspace : ToWorkspace  VariableName=innerCondAirTemp_inK  SampleTime=-1
  To Workspace1 : ToWorkspace  VariableName=innerCondAirTemp_outK  SampleTime=-1
  To Workspace2 : ToWorkspace  VariableName=airMassFlowRateCabin_in  SampleTime=-1
  C : PMIOPort  Side=Left
  B : PMIOPort  Port=2  Side=Left
  D : PMIOPort  Port=3  Side=Right
  A : PMIOPort  Port=4  Side=Right
  wires:
  PS-Simulink Converter/1 -> Scope2/1, To Workspace/1
  PS-Simulink Converter1/1 -> Scope1/1, To Workspace1/1
  PS-Simulink Converter2/1 -> Scope/1, To Workspace2/1
  connections:
  SR2/RConn1 -- B/RConn1
  SR1/LConn1 -- A/RConn1
  Inner Condenser/LConn1 -- SR1/RConn1
  Inner Condenser/LConn3 -- SR2/LConn1
  Inner Condenser/RConn3 -- C/RConn1 -- Pressure & Temperature Sensor (MA)/LConn1
  Inner Condenser/RConn1 -- Flow Rate Sensor (MA)/LConn1 -- Pressure & Temperature Sensor (MA)1/LConn1
  PS-Simulink Converter/LConn1 -- Pressure & Temperature Sensor (MA)/RConn1
  PS-Simulink Converter1/LConn1 -- Pressure & Temperature Sensor (MA)1/RConn1
  PS-Simulink Converter2/LConn1 -- Flow Rate Sensor (MA)/RConn2
  Flow Rate Sensor (MA)/RConn1 -- D/RConn1
